simulink model "sfGetStartedBreakpoints"  (R2025b)
settings: Solver=FixedStepAuto  StartTime=0.0  StopTime=100  FixedStep=1  RelTol=1e-3
settings Model: PacingRate=4  Creator=The MathWorks, Inc.  LastModifiedBy=The MathWorks, Inc.

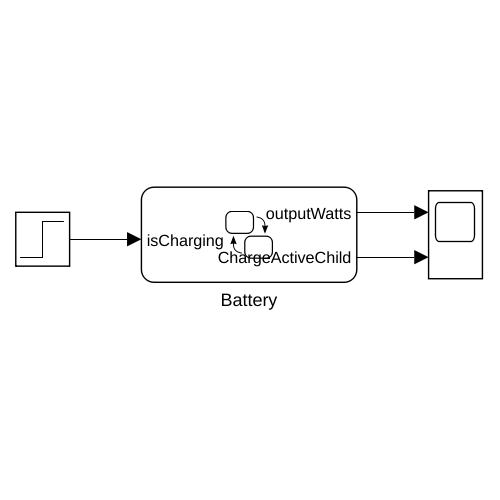
[thumbnail: Simulink's stored preview of the top-level diagram]
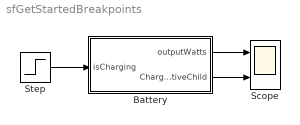
== system sfGetStartedBreakpoints ==
  Battery : Stateflow chart  TreatAsAtomicUnit=on
  Scope : Scope  NumInputPorts=2
      settings: ActiveDisplayYMinimum=-1  ActiveDisplayYMaximum=1
  Step : Step  Time=50  SampleTime=0
  wires:
  Step/1 -> Battery/1(isCharging)
  Battery/1(outputWatts) -> Scope/1
  Battery/2(ChargeActiveChild) -> Scope/2

== stateflow chart sfGetStartedBreakpoints/Battery ==
  state Charge
    entry:
    outputWatts=0;
    state FastCharge
      during:
      batteryLevel=batteryLevel+4;
    state SlowCharge
      during:
      batteryLevel=batteryLevel+1;
    state Full
    (default) -> FastCharge
    FastCharge -> SlowCharge : [batteryLevel>80]
    SlowCharge -> Full : [batteryLevel==100]
  state Discharge
    entry:
    outputWatts=4.5;
    state Powered
      during:
      batteryLevel=batteryLevel-3;
    state Empty
      entry:
      batteryLevel=0;
      outputWatts=0;
    (default) -> Powered
    Powered -> Empty : [batteryLevel<=0]
  (default) -> Charge
  Charge -> Discharge : after(1,sec)[isCharging]
  Discharge -> Charge : [~isCharging]
  data: isCharging input; outputWatts output; batteryLevel local =50; ChargeActiveChild output Enum: ChargeModeType
